simulink model "WarehouseFleetSim"  (R2024b)
settings: Solver=ode4  StartTime=0.0  StopTime=inf  FixedStep=0.02  RelTol=1e-3
StopFcn:
  | try, fleetVisionStep('close'); catch, end; try, phase3('stopped'); catch, end
model workspace (MAT data in the model file):
  HomePose1 = [-20 7.3 0]
  HomePose2 = [-20 3.6 0]
  HomePose3 = [-20 11 0]
  HomePose4 = [-24.5 3.6 0]
  HomePose5 = [-24.5 7.3 0]
  HomePose6 = [-24.5 11 0]
  Zero = 0
  gen3 : robotics.RigidBodyTree (value not decoded)
  qStow = [0; 0; 0.261799387799; 3.14159265359; -2.26892802759; 0; 0.959931088597; 1.57079632679]
undefined symbols (not defined in the file or in its folder): Actor, setupFleetScene, Sim3dSensor, World
libraries: sim3dlib x128, sim3dcameralib x7, robotmobilelib x6, robotsim3dlib x6
(part 4 of 4)

== stateflow chart WarehouseFleetSim/Robot 5/RobotTaskFSM ==
  settings: updateMethod=DISCRETE  sampleTime=0.02
  state IDLE
    en: TaskState=uint8(0); GoalX=-24.5000; GoalY=7.3000; GraspCmd=false; PlaceCmd=false;
  state NAV_TO_STAGING
    en: TaskState=uint8(1); GoalX=15.5000; GoalY=46.0556; GraspCmd=false; PlaceCmd=false;
  state DOCK_SHELF
    en: TaskState=uint8(10); GoalX=14.1900; GoalY=46.0556; IKTargetX=BoxX; IKTargetY=BoxY; IKTargetZ=BoxZ; GraspCmd=false; PlaceCmd=false;
  state ARM_EXTEND
    en: TaskState=uint8(2); IKTargetX=BoxX; IKTargetY=BoxY; IKTargetZ=BoxZ; GraspCmd=false;
  state GRASP
    en: TaskState=uint8(3); GraspCmd=true; PlaceCmd=false;
  state ARM_RETRACT
    en: TaskState=uint8(4); GraspCmd=true; PlaceCmd=false;
  state NAV_TO_TABLE
    en: TaskState=uint8(5); GoalX=18.5000; GoalY=65.1000; GraspCmd=true;
  state ARM_PLACE
    en: TaskState=uint8(6); IKTargetX=18.5000; IKTargetY=65.9700; IKTargetZ=1.0700; GraspCmd=true;
  state RELEASE
    en: TaskState=uint8(8); GraspCmd=false; PlaceCmd=true;
  state ARM_STOW
    en: TaskState=uint8(9); GraspCmd=false; PlaceCmd=false;
  state RETURN_HOME
    en: TaskState=uint8(7); GoalX=-24.5000; GoalY=7.3000; GraspCmd=false;
  state FAULT_HOLD
    en: TaskState=uint8(11); GraspCmd=false; PlaceCmd=false;
  state MISSION_DONE
    en: TaskState=uint8(12); GoalX=-24.5000; GoalY=7.3000; GraspCmd=false; PlaceCmd=false;
  NAV_TO_STAGING -> IDLE [order 2] : [AtGoal && ScanDone && ~PerceptionValid]
  RETURN_HOME -> IDLE : [AtGoal || MoreBoxes]
  (default) -> IDLE
  GRASP -> ARM_RETRACT [order 2] : [ArmDone && IsTargetGrasped]
  DOCK_SHELF -> FAULT_HOLD [order 2] : [ArmFault]
  ARM_EXTEND -> FAULT_HOLD [order 1] : [ArmFault]
  GRASP -> FAULT_HOLD [order 1] : [ArmFault]
  IDLE -> NAV_TO_STAGING [order 1] : after(1,sec)[MoreBoxes]
  NAV_TO_STAGING -> DOCK_SHELF [order 1] : [AtGoal && ScanDone && PerceptionValid]
  DOCK_SHELF -> ARM_EXTEND [order 1] : [AtGoal && ArmDone]
  ARM_EXTEND -> GRASP [order 2] : [ArmDone]
  IDLE -> MISSION_DONE [order 3] : after(2,sec)[~MoreBoxes && Finish && ~NeedHome]
  IDLE -> RETURN_HOME [order 2] : after(1,sec)[~MoreBoxes && NeedHome]
  FAULT_HOLD -> ARM_RETRACT [order 1] : [~ArmFault && IsTargetGrasped]
  ARM_RETRACT -> NAV_TO_TABLE [order 2] : [ArmDone]
  ARM_STOW -> RETURN_HOME : [ArmDone]
  NAV_TO_TABLE -> ARM_PLACE : [AtGoal]
  ARM_PLACE -> FAULT_HOLD [order 1] : [ArmFault]
  ARM_PLACE -> RELEASE [order 2] : [ArmDone]
  FAULT_HOLD -> ARM_STOW [order 2] : [~ArmFault && ~IsTargetGrasped]
  RELEASE -> ARM_STOW [order 1] : [~IsTargetGrasped]
  RELEASE -> ARM_STOW [order 2] : after(1,sec)
  ARM_RETRACT -> FAULT_HOLD [order 1] : [ArmFault]
  data: AtGoal input boolean; ArmDone input boolean; PerceptionValid input boolean; BoxX input double; BoxY input double; BoxZ input double; IsTargetGrasped input boolean; ArmFault input boolean; MoreBoxes input boolean; ScanDone input boolean; Finish input boolean; NeedHome input boolean; TaskState output uint8; GoalX output double; GoalY output double; IKTargetX output double; IKTargetY output double; IKTargetZ output double; GraspCmd output boolean; PlaceCmd output boolean

== matlab function WarehouseFleetSim/Robot 5/Idx Select ==
  data: c2 input; idx output
function idx = fcn(c2)
idx = c2(1);

== matlab function WarehouseFleetSim/Robot 5/Box Meas Pick ==
  data: pool input; y output; idx input
function y = fcn(pool,idx)
y = zeros(1,9); i = round(idx);
if i>=1 && i<=54, y(1:3) = pool(3*i-2:3*i); end

== matlab function WarehouseFleetSim/Robot 5/Robot Pack ==
  data: c input; y output; r input; d input; c2 input
function y = fcn(c,r,d,c2)
y = [c r double(d) c2(1)];

== matlab function WarehouseFleetSim/Robot 5/Lift Select ==
  data: q input; y output
function y = fcn(q)
y = q(1);

== matlab function WarehouseFleetSim/Robot 1/Idx Select ==
  data: c2 input; idx output
function idx = fcn(c2)
idx = c2(1);

== matlab function WarehouseFleetSim/Robot 5/Pose To Robot Transform ==
  data: pose input; translation output; rotation output
function [translation,rotation] = fcn(pose)
translation = [pose(1), pose(2), 0];
rotation = [pose(3), 0, 0];

== stateflow chart WarehouseFleetSim/Robot 6/RobotTaskFSM ==
  settings: updateMethod=DISCRETE  sampleTime=0.02
  state IDLE
    en: TaskState=uint8(0); GoalX=-24.5000; GoalY=11.0000; GraspCmd=false; PlaceCmd=false;
  state NAV_TO_STAGING
    en: TaskState=uint8(1); GoalX=15.5000; GoalY=46.0556; GraspCmd=false; PlaceCmd=false;
  state DOCK_SHELF
    en: TaskState=uint8(10); GoalX=14.1900; GoalY=46.0556; IKTargetX=BoxX; IKTargetY=BoxY; IKTargetZ=BoxZ; GraspCmd=false; PlaceCmd=false;
  state ARM_EXTEND
    en: TaskState=uint8(2); IKTargetX=BoxX; IKTargetY=BoxY; IKTargetZ=BoxZ; GraspCmd=false;
  state GRASP
    en: TaskState=uint8(3); GraspCmd=true; PlaceCmd=false;
  state ARM_RETRACT
    en: TaskState=uint8(4); GraspCmd=true; PlaceCmd=false;
  state NAV_TO_TABLE
    en: TaskState=uint8(5); GoalX=18.5000; GoalY=65.1000; GraspCmd=true;
  state ARM_PLACE
    en: TaskState=uint8(6); IKTargetX=18.5000; IKTargetY=65.9700; IKTargetZ=1.0700; GraspCmd=true;
  state RELEASE
    en: TaskState=uint8(8); GraspCmd=false; PlaceCmd=true;
  state ARM_STOW
    en: TaskState=uint8(9); GraspCmd=false; PlaceCmd=false;
  state RETURN_HOME
    en: TaskState=uint8(7); GoalX=-24.5000; GoalY=11.0000; GraspCmd=false;
  state FAULT_HOLD
    en: TaskState=uint8(11); GraspCmd=false; PlaceCmd=false;
  state MISSION_DONE
    en: TaskState=uint8(12); GoalX=-24.5000; GoalY=11.0000; GraspCmd=false; PlaceCmd=false;
  NAV_TO_STAGING -> IDLE [order 2] : [AtGoal && ScanDone && ~PerceptionValid]
  RETURN_HOME -> IDLE : [AtGoal || MoreBoxes]
  (default) -> IDLE
  GRASP -> ARM_RETRACT [order 2] : [ArmDone && IsTargetGrasped]
  DOCK_SHELF -> FAULT_HOLD [order 2] : [ArmFault]
  ARM_EXTEND -> FAULT_HOLD [order 1] : [ArmFault]
  GRASP -> FAULT_HOLD [order 1] : [ArmFault]
  IDLE -> NAV_TO_STAGING [order 1] : after(1,sec)[MoreBoxes]
  NAV_TO_STAGING -> DOCK_SHELF [order 1] : [AtGoal && ScanDone && PerceptionValid]
  DOCK_SHELF -> ARM_EXTEND [order 1] : [AtGoal && ArmDone]
  ARM_EXTEND -> GRASP [order 2] : [ArmDone]
  IDLE -> MISSION_DONE [order 3] : after(2,sec)[~MoreBoxes && Finish && ~NeedHome]
  IDLE -> RETURN_HOME [order 2] : after(1,sec)[~MoreBoxes && NeedHome]
  FAULT_HOLD -> ARM_RETRACT [order 1] : [~ArmFault && IsTargetGrasped]
  ARM_RETRACT -> NAV_TO_TABLE [order 2] : [ArmDone]
  ARM_STOW -> RETURN_HOME : [ArmDone]
  NAV_TO_TABLE -> ARM_PLACE : [AtGoal]
  ARM_PLACE -> FAULT_HOLD [order 1] : [ArmFault]
  ARM_PLACE -> RELEASE [order 2] : [ArmDone]
  FAULT_HOLD -> ARM_STOW [order 2] : [~ArmFault && ~IsTargetGrasped]
  RELEASE -> ARM_STOW [order 1] : [~IsTargetGrasped]
  RELEASE -> ARM_STOW [order 2] : after(1,sec)
  ARM_RETRACT -> FAULT_HOLD [order 1] : [ArmFault]
  data: AtGoal input boolean; ArmDone input boolean; PerceptionValid input boolean; BoxX input double; BoxY input double; BoxZ input double; IsTargetGrasped input boolean; ArmFault input boolean; MoreBoxes input boolean; ScanDone input boolean; Finish input boolean; NeedHome input boolean; TaskState output uint8; GoalX output double; GoalY output double; IKTargetX output double; IKTargetY output double; IKTargetZ output double; GraspCmd output boolean; PlaceCmd output boolean

== matlab function WarehouseFleetSim/Robot 6/Idx Select ==
  data: c2 input; idx output
function idx = fcn(c2)
idx = c2(1);

== matlab function WarehouseFleetSim/Pool Pack ==
  data: a1 input; y output; a2 input; a3 input; a4 input; a5 input; a6 input; a7 input; a8 input; a9 input; a10 input; a11 input; a12 input; a13 input; a14 input; a15 input; a16 input; a17 input; a18 input; a19 input; a20 input; a21 input; a22 input; a23 input; a24 input; a25 input; a26 input; a27 input; a28 input; a29 input; a30 input; a31 input; a32 input; a33 input; a34 input; a35 input; a36 input; a37 input; a38 input; a39 input; a40 input; a41 input; a42 input; a43 input; a44 input; a45 input; a46 input; a47 input; a48 input; a49 input; a50 input; a51 input; a52 input; a53 input; a54 input
function y = fcn(a1,a2,a3,a4,a5,a6,a7,a8,a9,a10,a11,a12,a13,a14,a15,a16,a17,a18,a19,a20,a21,a22,a23,a24,a25,a26,a27,a28,a29,a30,a31,a32,a33,a34,a35,a36,a37,a38,a39,a40,a41,a42,a43,a44,a45,a46,a47,a48,a49,a50,a51,a52,a53,a54)
y = [reshape(a1,1,[]) reshape(a2,1,[]) reshape(a3,1,[]) reshape(a4,1,[]) reshape(a5,1,[]) reshape(a6,1,[]) reshape(a7,1,[]) reshape(a8,1,[]) reshape(a9,1,[]) reshape(a10,1,[]) reshape(a11,1,[]) reshape(a12,1,[]) reshape(a13,1,[]) reshape(a14,1,[]) reshape(a15,1,[]) reshape(a16,1,[]) reshape(a17,1,[]) reshape(a18,1,[]) reshape(a19,1,[]) reshape(a20,1,[]) reshape(a21,1,[]) reshape(a22,1,[]) reshape(a23,1,[]) reshape(a24,1,[]) reshape(a25,1,[]) reshape(a26,1,[]) reshape(a27,1,[]) reshape(a28,1,[]) reshape(a29,1,[]) reshape(a30,1,[]) reshape(a31,1,[]) reshape(a32,1,[]) reshape(a33,1,[]) reshape(a34,1,[]) reshape(a35,1,[]) reshape(a36,1,[]) reshape(a37,1,[]) reshape(a38,1,[]) reshape(a39,1,[]) reshape(a40,1,[]) reshape(a41,1,[]) reshape(a42,1,[]) reshape(a43,1,[]) reshape(a44,1,[]) reshape(a45,1,[]) reshape(a46,1,[]) reshape(a47,1,[]) reshape(a48,1,[]) reshape(a49,1,[]) reshape(a50,1,[]) reshape(a51,1,[]) reshape(a52,1,[]) reshape(a53,1,[]) reshape(a54,1,[])];

== matlab function WarehouseFleetSim/Robot 6/Box Meas Pick ==
  data: pool input; y output; idx input
function y = fcn(pool,idx)
y = zeros(1,9); i = round(idx);
if i>=1 && i<=54, y(1:3) = pool(3*i-2:3*i); end

== matlab function WarehouseFleetSim/Robot 6/Robot Pack ==
  data: c input; y output; r input; d input; c2 input
function y = fcn(c,r,d,c2)
y = [c r double(d) c2(1)];

== matlab function WarehouseFleetSim/Robot 6/Lift Select ==
  data: q input; y output
function y = fcn(q)
y = q(1);

== matlab function WarehouseFleetSim/Robot 6/Pose To Robot Transform ==
  data: pose input; translation output; rotation output
function [translation,rotation] = fcn(pose)
translation = [pose(1), pose(2), 0];
rotation = [pose(3), 0, 0];

== matlab function WarehouseFleetSim/Robot 1 Cam Pose ==
  data: pose input; translation output; lift input; rotation output
function [translation,rotation] = fcn(pose,lift)
yaw=pose(3); c=cos(yaw); s=sin(yaw);
f=0.2; l=0; z=1.37+lift;
translation=[pose(1)+f*c-l*s pose(2)+f*s+l*c z];
rotation=[0 22 yaw*180/pi];

== matlab function WarehouseFleetSim/Robot 2 Cam Pose ==
  data: pose input; translation output; lift input; rotation output
function [translation,rotation] = fcn(pose,lift)
yaw=pose(3); c=cos(yaw); s=sin(yaw);
f=0.2; l=0; z=1.37+lift;
translation=[pose(1)+f*c-l*s pose(2)+f*s+l*c z];
rotation=[0 22 yaw*180/pi];

== matlab function WarehouseFleetSim/Robot 3 Cam Pose ==
  data: pose input; translation output; lift input; rotation output
function [translation,rotation] = fcn(pose,lift)
yaw=pose(3); c=cos(yaw); s=sin(yaw);
f=0.2; l=0; z=1.37+lift;
translation=[pose(1)+f*c-l*s pose(2)+f*s+l*c z];
rotation=[0 22 yaw*180/pi];

== matlab function WarehouseFleetSim/Robot 4 Cam Pose ==
  data: pose input; translation output; lift input; rotation output
function [translation,rotation] = fcn(pose,lift)
yaw=pose(3); c=cos(yaw); s=sin(yaw);
f=0.2; l=0; z=1.37+lift;
translation=[pose(1)+f*c-l*s pose(2)+f*s+l*c z];
rotation=[0 22 yaw*180/pi];

== matlab function WarehouseFleetSim/Robot 5 Cam Pose ==
  data: pose input; translation output; lift input; rotation output
function [translation,rotation] = fcn(pose,lift)
yaw=pose(3); c=cos(yaw); s=sin(yaw);
f=0.2; l=0; z=1.37+lift;
translation=[pose(1)+f*c-l*s pose(2)+f*s+l*c z];
rotation=[0 22 yaw*180/pi];

== matlab function WarehouseFleetSim/Robot 6 Cam Pose ==
  data: pose input; translation output; lift input; rotation output
function [translation,rotation] = fcn(pose,lift)
yaw=pose(3); c=cos(yaw); s=sin(yaw);
f=0.2; l=0; z=1.37+lift;
translation=[pose(1)+f*c-l*s pose(2)+f*s+l*c z];
rotation=[0 22 yaw*180/pi];

== matlab function WarehouseFleetSim/Carton Router ==
  data: p1 input; trans output; p2 input; p3 input; p4 input; p5 input; p6 input; fc input; fr input; fa input; rot output; drv output
function [trans,rot,drv] = fcn(p1,p2,p3,p4,p5,p6,fc,fr,fa)
% every robot sends [carton(1x3) rot(1x3) drive idx]; the fleet block sends park / arrival commands. A robot that drives carton j beats the fleet.
M=54; trans=fc; rot=fr; drv=(fa>0.5);
P=[p1;p2;p3;p4;p5;p6];
for r=1:6
  j=round(P(r,8));
  if j>=1 && j<=M && P(r,7)>0.5
    trans(3*j-2:3*j)=P(r,1:3); rot(3*j-2:3*j)=P(r,4:6); drv(j)=true;
  end
end

== matlab function WarehouseFleetSim/Marker 1 Calc ==
  data: pose input; t1 output; r1 output; t2 output; r2 output; t3 output; r3 output
function [t1,r1,t2,r2,t3,r3] = fcn(pose)
% slat q sits at body angle (pi + th) on the chassis radius; its thin axis is radial.  Unreal frame: y negated, yaw negated.
R=0.3380; z=0.200; th=[-0.2618 0 0.2618];
p=zeros(3,3); r=zeros(3,3);
for q=1:3
  f=pose(3)+pi+th(q); p(q,:)=[pose(1)+R*cos(f) -(pose(2)+R*sin(f)) z]; r(q,:)=[0 0 -f];
end
t1=p(1,:); r1=r(1,:); t2=p(2,:); r2=r(2,:); t3=p(3,:); r3=r(3,:);

== matlab function WarehouseFleetSim/Marker 2 Calc ==
  data: pose input; t1 output; r1 output; t2 output; r2 output; t3 output; r3 output
function [t1,r1,t2,r2,t3,r3] = fcn(pose)
% slat q sits at body angle (pi + th) on the chassis radius; its thin axis is radial.  Unreal frame: y negated, yaw negated.
R=0.3380; z=0.200; th=[-0.2618 0 0.2618];
p=zeros(3,3); r=zeros(3,3);
for q=1:3
  f=pose(3)+pi+th(q); p(q,:)=[pose(1)+R*cos(f) -(pose(2)+R*sin(f)) z]; r(q,:)=[0 0 -f];
end
t1=p(1,:); r1=r(1,:); t2=p(2,:); r2=r(2,:); t3=p(3,:); r3=r(3,:);

== matlab function WarehouseFleetSim/Marker 3 Calc ==
  data: pose input; t1 output; r1 output; t2 output; r2 output; t3 output; r3 output
function [t1,r1,t2,r2,t3,r3] = fcn(pose)
% slat q sits at body angle (pi + th) on the chassis radius; its thin axis is radial.  Unreal frame: y negated, yaw negated.
R=0.3380; z=0.200; th=[-0.2618 0 0.2618];
p=zeros(3,3); r=zeros(3,3);
for q=1:3
  f=pose(3)+pi+th(q); p(q,:)=[pose(1)+R*cos(f) -(pose(2)+R*sin(f)) z]; r(q,:)=[0 0 -f];
end
t1=p(1,:); r1=r(1,:); t2=p(2,:); r2=r(2,:); t3=p(3,:); r3=r(3,:);

== matlab function WarehouseFleetSim/Marker 4 Calc ==
  data: pose input; t1 output; r1 output; t2 output; r2 output; t3 output; r3 output
function [t1,r1,t2,r2,t3,r3] = fcn(pose)
% slat q sits at body angle (pi + th) on the chassis radius; its thin axis is radial.  Unreal frame: y negated, yaw negated.
R=0.3380; z=0.200; th=[-0.2618 0 0.2618];
p=zeros(3,3); r=zeros(3,3);
for q=1:3
  f=pose(3)+pi+th(q); p(q,:)=[pose(1)+R*cos(f) -(pose(2)+R*sin(f)) z]; r(q,:)=[0 0 -f];
end
t1=p(1,:); r1=r(1,:); t2=p(2,:); r2=r(2,:); t3=p(3,:); r3=r(3,:);

== matlab function WarehouseFleetSim/Marker 5 Calc ==
  data: pose input; t1 output; r1 output; t2 output; r2 output; t3 output; r3 output
function [t1,r1,t2,r2,t3,r3] = fcn(pose)
% slat q sits at body angle (pi + th) on the chassis radius; its thin axis is radial.  Unreal frame: y negated, yaw negated.
R=0.3380; z=0.200; th=[-0.2618 0 0.2618];
p=zeros(3,3); r=zeros(3,3);
for q=1:3
  f=pose(3)+pi+th(q); p(q,:)=[pose(1)+R*cos(f) -(pose(2)+R*sin(f)) z]; r(q,:)=[0 0 -f];
end
t1=p(1,:); r1=r(1,:); t2=p(2,:); r2=r(2,:); t3=p(3,:); r3=r(3,:);

== matlab function WarehouseFleetSim/Marker 6 Calc ==
  data: pose input; t1 output; r1 output; t2 output; r2 output; t3 output; r3 output
function [t1,r1,t2,r2,t3,r3] = fcn(pose)
% slat q sits at body angle (pi + th) on the chassis radius; its thin axis is radial.  Unreal frame: y negated, yaw negated.
R=0.3380; z=0.200; th=[-0.2618 0 0.2618];
p=zeros(3,3); r=zeros(3,3);
for q=1:3
  f=pose(3)+pi+th(q); p(q,:)=[pose(1)+R*cos(f) -(pose(2)+R*sin(f)) z]; r(q,:)=[0 0 -f];
end
t1=p(1,:); r1=r(1,:); t2=p(2,:); r2=r(2,:); t3=p(3,:); r3=r(3,:);

== matlab function WarehouseFleetSim/Poses Mux ==
  data: a1 input; y output; a2 input; a3 input; a4 input; a5 input; a6 input
function y = fcn(a1,a2,a3,a4,a5,a6)
y = [reshape(a1,1,3) reshape(a2,1,3) reshape(a3,1,3) reshape(a4,1,3) reshape(a5,1,3) reshape(a6,1,3)];

== matlab function WarehouseFleetSim/Lifts Mux ==
  data: a1 input; y output; a2 input; a3 input; a4 input; a5 input; a6 input
function y = fcn(a1,a2,a3,a4,a5,a6)
y = [a1(1) a2(1) a3(1) a4(1) a5(1) a6(1)];

== matlab function WarehouseFleetSim/Fleet Camera Pose ==
  data: poses input; translation output; lifts input; rotation output; selPose output; selLift output; sel output
function [translation,rotation,selPose,selLift,sel] = fcn(poses,lifts)
coder.extrinsic('phase3SelRobot');
sel=1; sel=phase3SelRobot();
sel=min(max(round(sel),1),6);
selPose=poses(3*sel-2:3*sel); selLift=lifts(sel);
yaw=selPose(3); c=cos(yaw); s=sin(yaw);
f=0.2; l=0; z=1.37+selLift;
translation=[selPose(1)+f*c-l*s selPose(2)+f*s+l*c z];
rotation=[0 22 yaw*180/pi];

== matlab function WarehouseFleetSim/Fleet Vision Viewer ==
  data: img input; ok output; pose input; lift input; sel input
function ok = fcn(img,pose,lift,sel)
coder.extrinsic('fleetVisionStep');
fleetVisionStep(img,pose,lift,sel);
ok=uint8(0);
